simulink model "Koudruped_simcape"  (R2025b)
settings: Solver=VariableStepAuto  StartTime=0.0  StopTime=30  RelTol=1e-2
undefined symbols (not defined in the file or in its folder): fractalcoef, smiData, X, Y, Z
libraries: sm_lib x589, nesl_utility x93, slpidlib x5, mspsensorlib x4, simulink_extras x4, mspfiltlib x3, simulink x2
(part 15 of 16)

== system Koudruped_simcape/quad_step_1_RIGID/govde_step_1_RIGID/A_0002_A_GovdeUst_v11_step_1_RIGID ==
  ReferenceFrame : sm_lib/Frames and Transforms/Reference Frame
  Solid : sm_lib/Body Elements/File Solid  ExtGeomFileName=A-0002-A_GovdeUst v11.step_Varsayılan_sldprt.STEP  UnitType=FromFile  ExtGeomFileUnits=m  StepReaderType=HEX  ExportConvexHullGeometry=off  InertiaType=Custom  BasedOnType=DensityFromFile  Density=1000  DensityUnits=kg/m^3  Mass=smiData.Solid(4).mass  MassUnits=kg  CenterOfMass=smiData.Solid(4).CoM  CenterOfMassUnits=mm  MomentsOfInertia=smiData.Solid(4).MoI  MomentsOfInertiaUnits=kg*mm^2  ProductsOfInertia=smiData.Solid(4).PoI  ProductsOfInertiaUnits=kg*mm^2  GraphicType=FromGeometry  MarkerShape=Sphere  MarkerSize=10  GraphicVisPropType=SimpleVisualProperties  GraphicDiffuseColor=smiData.Solid(4).color  GraphicOpacity=smiData.Solid(4).opacity  GraphicSpecularColor=[0.5 0.5 0.5 1.0]  GraphicAmbientColor=[0.15 0.15 0.15 1.0]  GraphicEmissiveColor=[0.0 0.0 0.0 1.0]  GraphicShininess=75  DoExposeReferenceFrame=on  SerializedFrames=<Frames/>
  F : PMIOPort  Side=Left
  connections:
  ReferenceFrame/RConn1 -- Solid/RConn1 -- F/RConn1

== system Koudruped_simcape/quad_step_1_RIGID/govde_step_1_RIGID/Arms_step_1_RIGID ==
  ReferenceFrame : sm_lib/Frames and Transforms/Reference Frame
  Transform : sm_lib/Frames and Transforms/Rigid Transform  RotationMethod=ArbitraryAxis  FollAlignAxisA=+X  BaseAlignAxisA=+Y  FollAlignAxisB=+Y  BaseAlignAxisB=+Z  RotationStandardAxis=+Z  RotationAngle=smiData.RigidTransform(1).angle  RotationAngleUnits=rad  RotationArbitraryAxis=smiData.RigidTransform(1).axis  RotationSequenceAxes=FollowerAxes  RotationSequence=XYX  RotationSequenceAngles=[0 0 0]  RotationSequenceAnglesUnits=deg  RotationMatrix=[1 0 0;0 1 0;0 0 1]  Quaternion=[1 0 0 0]  TranslationMethod=Cartesian  TranslationCartesianOffset=smiData.RigidTransform(1).translation  TranslationCartesianOffsetUnits=mm  TranslationStandardAxis=+Z  TranslationStandardOffset=0  TranslationStandardOffsetUnits=m  TranslationROffset=0  TranslationROffsetUnits=m  TranslationThetaOffset=0  TranslationThetaOffsetUnits=deg  TranslationZOffset=0  TranslationZOffsetUnits=m
  Transform1 : sm_lib/Frames and Transforms/Rigid Transform  RotationMethod=ArbitraryAxis  FollAlignAxisA=+X  BaseAlignAxisA=+Y  FollAlignAxisB=+Y  BaseAlignAxisB=+Z  RotationStandardAxis=+Z  RotationAngle=smiData.RigidTransform(2).angle  RotationAngleUnits=rad  RotationArbitraryAxis=smiData.RigidTransform(2).axis  RotationSequenceAxes=FollowerAxes  RotationSequence=XYX  RotationSequenceAngles=[0 0 0]  RotationSequenceAnglesUnits=deg  RotationMatrix=[1 0 0;0 1 0;0 0 1]  Quaternion=[1 0 0 0]  TranslationMethod=Cartesian  TranslationCartesianOffset=smiData.RigidTransform(2).translation  TranslationCartesianOffsetUnits=mm  TranslationStandardAxis=+Z  TranslationStandardOffset=0  TranslationStandardOffsetUnits=m  TranslationROffset=0  TranslationROffsetUnits=m  TranslationThetaOffset=0  TranslationThetaOffsetUnits=deg  TranslationZOffset=0  TranslationZOffsetUnits=m
  arm_step_1_RIGID : Subsystem
  F : PMIOPort  Side=Left
  connections:
  Transform/RConn1 -- arm_step_1_RIGID/LConn1
  ReferenceFrame/RConn1 -- Transform/LConn1 -- Transform1/RConn1
  Transform1/LConn1 -- F/RConn1

== system Koudruped_simcape/quad_step_1_RIGID/govde_step_1_RIGID/Eklemler_step_1_RIGID ==
  A_0005_AC_ServoYatagi_sol_v15_step_1_RIGID : Subsystem
  ReferenceFrame : sm_lib/Frames and Transforms/Reference Frame
  Transform : sm_lib/Frames and Transforms/Rigid Transform  RotationMethod=ArbitraryAxis  FollAlignAxisA=+X  BaseAlignAxisA=+Y  FollAlignAxisB=+Y  BaseAlignAxisB=+Z  RotationStandardAxis=+Z  RotationAngle=smiData.RigidTransform(3).angle  RotationAngleUnits=rad  RotationArbitraryAxis=smiData.RigidTransform(3).axis  RotationSequenceAxes=FollowerAxes  RotationSequence=XYX  RotationSequenceAngles=[0 0 0]  RotationSequenceAnglesUnits=deg  RotationMatrix=[1 0 0;0 1 0;0 0 1]  Quaternion=[1 0 0 0]  TranslationMethod=Cartesian  TranslationCartesianOffset=smiData.RigidTransform(3).translation  TranslationCartesianOffsetUnits=mm  TranslationStandardAxis=+Z  TranslationStandardOffset=0  TranslationStandardOffsetUnits=m  TranslationROffset=0  TranslationROffsetUnits=m  TranslationThetaOffset=0  TranslationThetaOffsetUnits=deg  TranslationZOffset=0  TranslationZOffsetUnits=m
  Transform1 : sm_lib/Frames and Transforms/Rigid Transform  RotationMethod=ArbitraryAxis  FollAlignAxisA=+X  BaseAlignAxisA=+Y  FollAlignAxisB=+Y  BaseAlignAxisB=+Z  RotationStandardAxis=+Z  RotationAngle=smiData.RigidTransform(4).angle  RotationAngleUnits=rad  RotationArbitraryAxis=smiData.RigidTransform(4).axis  RotationSequenceAxes=FollowerAxes  RotationSequence=XYX  RotationSequenceAngles=[0 0 0]  RotationSequenceAnglesUnits=deg  RotationMatrix=[1 0 0;0 1 0;0 0 1]  Quaternion=[1 0 0 0]  TranslationMethod=Cartesian  TranslationCartesianOffset=smiData.RigidTransform(4).translation  TranslationCartesianOffsetUnits=mm  TranslationStandardAxis=+Z  TranslationStandardOffset=0  TranslationStandardOffsetUnits=m  TranslationROffset=0  TranslationROffsetUnits=m  TranslationThetaOffset=0  TranslationThetaOffsetUnits=deg  TranslationZOffset=0  TranslationZOffsetUnits=m
  F : PMIOPort  Side=Left
  connections:
  A_0005_AC_ServoYatagi_sol_v15_step_1_RIGID/LConn1 -- Transform/RConn1
  ReferenceFrame/RConn1 -- Transform/LConn1 -- Transform1/RConn1
  Transform1/LConn1 -- F/RConn1

== system Koudruped_simcape/quad_step_1_RIGID/ön takım/ön takım ==
  ReferenceFrame : sm_lib/Frames and Transforms/Reference Frame
  Transform : sm_lib/Frames and Transforms/Rigid Transform  RotationMethod=ArbitraryAxis  FollAlignAxisA=+X  BaseAlignAxisA=+Y  FollAlignAxisB=+Y  BaseAlignAxisB=+Z  RotationStandardAxis=+Z  RotationAngle=smiData.RigidTransform(8).angle  RotationAngleUnits=rad  RotationArbitraryAxis=smiData.RigidTransform(8).axis  RotationSequenceAxes=FollowerAxes  RotationSequence=XYX  RotationSequenceAngles=[0 0 0]  RotationSequenceAnglesUnits=deg  RotationMatrix=[1 0 0;0 1 0;0 0 1]  Quaternion=[1 0 0 0]  TranslationMethod=Cartesian  TranslationCartesianOffset=smiData.RigidTransform(8).translation  TranslationCartesianOffsetUnits=mm  TranslationStandardAxis=+Z  TranslationStandardOffset=0  TranslationStandardOffsetUnits=m  TranslationROffset=0  TranslationROffsetUnits=m  TranslationThetaOffset=0  TranslationThetaOffsetUnits=deg  TranslationZOffset=0  TranslationZOffsetUnits=m
  Transform1 : sm_lib/Frames and Transforms/Rigid Transform  RotationMethod=ArbitraryAxis  FollAlignAxisA=+X  BaseAlignAxisA=+Y  FollAlignAxisB=+Y  BaseAlignAxisB=+Z  RotationStandardAxis=+Z  RotationAngle=smiData.RigidTransform(9).angle  RotationAngleUnits=rad  RotationArbitraryAxis=smiData.RigidTransform(9).axis  RotationSequenceAxes=FollowerAxes  RotationSequence=XYX  RotationSequenceAngles=[0 0 0]  RotationSequenceAnglesUnits=deg  RotationMatrix=[1 0 0;0 1 0;0 0 1]  Quaternion=[1 0 0 0]  TranslationMethod=Cartesian  TranslationCartesianOffset=smiData.RigidTransform(9).translation  TranslationCartesianOffsetUnits=mm  TranslationStandardAxis=+Z  TranslationStandardOffset=0  TranslationStandardOffsetUnits=m  TranslationROffset=0  TranslationROffsetUnits=m  TranslationThetaOffset=0  TranslationThetaOffsetUnits=deg  TranslationZOffset=0  TranslationZOffsetUnits=m
  Transform2 : sm_lib/Frames and Transforms/Rigid Transform  RotationMethod=ArbitraryAxis  FollAlignAxisA=+X  BaseAlignAxisA=+Y  FollAlignAxisB=+Y  BaseAlignAxisB=+Z  RotationStandardAxis=+Z  RotationAngle=smiData.RigidTransform(10).angle  RotationAngleUnits=rad  RotationArbitraryAxis=smiData.RigidTransform(10).axis  RotationSequenceAxes=FollowerAxes  RotationSequence=XYX  RotationSequenceAngles=[0 0 0]  RotationSequenceAnglesUnits=deg  RotationMatrix=[1 0 0;0 1 0;0 0 1]  Quaternion=[1 0 0 0]  TranslationMethod=Cartesian  TranslationCartesianOffset=smiData.RigidTransform(10).translation  TranslationCartesianOffsetUnits=mm  TranslationStandardAxis=+Z  TranslationStandardOffset=0  TranslationStandardOffsetUnits=m  TranslationROffset=0  TranslationROffsetUnits=m  TranslationThetaOffset=0  TranslationThetaOffsetUnits=deg  TranslationZOffset=0  TranslationZOffsetUnits=m
  Transform3 : sm_lib/Frames and Transforms/Rigid Transform  RotationMethod=ArbitraryAxis  FollAlignAxisA=+X  BaseAlignAxisA=+Y  FollAlignAxisB=+Y  BaseAlignAxisB=+Z  RotationStandardAxis=+Z  RotationAngle=smiData.RigidTransform(11).angle  RotationAngleUnits=rad  RotationArbitraryAxis=smiData.RigidTransform(11).axis  RotationSequenceAxes=FollowerAxes  RotationSequence=XYX  RotationSequenceAngles=[0 0 0]  RotationSequenceAnglesUnits=deg  RotationMatrix=[1 0 0;0 1 0;0 0 1]  Quaternion=[1 0 0 0]  TranslationMethod=Cartesian  TranslationCartesianOffset=smiData.RigidTransform(11).translation  TranslationCartesianOffsetUnits=mm  TranslationStandardAxis=+Z  TranslationStandardOffset=0  TranslationStandardOffsetUnits=m  TranslationROffset=0  TranslationROffsetUnits=m  TranslationThetaOffset=0  TranslationThetaOffsetUnits=deg  TranslationZOffset=0  TranslationZOffsetUnits=m
  arm_v2_1_step_1_RIGID : Subsystem
  ön alt : Subsystem
  ön üst : Subsystem
  F : PMIOPort  Side=Left
  connections:
  ön alt/LConn1 -- Transform/RConn1
  Transform1/RConn1 -- arm_v2_1_step_1_RIGID/LConn1
  Transform2/RConn1 -- ön üst/LConn1
  ReferenceFrame/RConn1 -- Transform1/LConn1 -- Transform2/LConn1 -- Transform/LConn1 -- Transform3/RConn1
  Transform3/LConn1 -- F/RConn1

== system Koudruped_simcape/quad_step_1_RIGID/govde_step_1_RIGID/Arms_step_1_RIGID/arm_step_1_RIGID ==
  ReferenceFrame : sm_lib/Frames and Transforms/Reference Frame
  Solid : sm_lib/Body Elements/File Solid  ExtGeomFileName=arm.step_Varsayılan_sldprt.STEP  UnitType=FromFile  ExtGeomFileUnits=m  StepReaderType=HEX  ExportConvexHullGeometry=off  InertiaType=Custom  BasedOnType=DensityFromFile  Density=1000  DensityUnits=kg/m^3  Mass=smiData.Solid(1).mass  MassUnits=kg  CenterOfMass=smiData.Solid(1).CoM  CenterOfMassUnits=mm  MomentsOfInertia=smiData.Solid(1).MoI  MomentsOfInertiaUnits=kg*mm^2  ProductsOfInertia=smiData.Solid(1).PoI  ProductsOfInertiaUnits=kg*mm^2  GraphicType=FromGeometry  MarkerShape=Sphere  MarkerSize=10  GraphicVisPropType=SimpleVisualProperties  GraphicDiffuseColor=smiData.Solid(1).color  GraphicOpacity=smiData.Solid(1).opacity  GraphicSpecularColor=[0.5 0.5 0.5 1.0]  GraphicAmbientColor=[0.15 0.15 0.15 1.0]  GraphicEmissiveColor=[0.0 0.0 0.0 1.0]  GraphicShininess=75  DoExposeReferenceFrame=on  SerializedFrames=<Frames/>
  F : PMIOPort  Side=Left
  connections:
  ReferenceFrame/RConn1 -- Solid/RConn1 -- F/RConn1

== system Koudruped_simcape/quad_step_1_RIGID/govde_step_1_RIGID/Eklemler_step_1_RIGID/A_0005_AC_ServoYatagi_sol_v15_step_1_RIGID ==
  ReferenceFrame : sm_lib/Frames and Transforms/Reference Frame
  Solid : sm_lib/Body Elements/File Solid  ExtGeomFileName=A_0005_AC_ServoYatagi_sol v15.step_Varsayılan_sldprt.STEP  UnitType=FromFile  ExtGeomFileUnits=m  StepReaderType=HEX  ExportConvexHullGeometry=off  InertiaType=Custom  BasedOnType=DensityFromFile  Density=1000  DensityUnits=kg/m^3  Mass=smiData.Solid(2).mass  MassUnits=kg  CenterOfMass=smiData.Solid(2).CoM  CenterOfMassUnits=mm  MomentsOfInertia=smiData.Solid(2).MoI  MomentsOfInertiaUnits=kg*mm^2  ProductsOfInertia=smiData.Solid(2).PoI  ProductsOfInertiaUnits=kg*mm^2  GraphicType=FromGeometry  MarkerShape=Sphere  MarkerSize=10  GraphicVisPropType=SimpleVisualProperties  GraphicDiffuseColor=smiData.Solid(2).color  GraphicOpacity=smiData.Solid(2).opacity  GraphicSpecularColor=[0.5 0.5 0.5 1.0]  GraphicAmbientColor=[0.15 0.15 0.15 1.0]  GraphicEmissiveColor=[0.0 0.0 0.0 1.0]  GraphicShininess=75  DoExposeReferenceFrame=on  SerializedFrames=<Frames/>
  F : PMIOPort  Side=Left
  connections:
  ReferenceFrame/RConn1 -- Solid/RConn1 -- F/RConn1

== system Koudruped_simcape/quad_step_1_RIGID/ön takım/ön takım/arm_v2_1_step_1_RIGID ==
  ReferenceFrame : sm_lib/Frames and Transforms/Reference Frame
  Solid : sm_lib/Body Elements/File Solid  ExtGeomFileName=arm v2 (1).step_Varsayılan_sldprt.STEP  UnitType=FromFile  ExtGeomFileUnits=m  StepReaderType=HEX  ExportConvexHullGeometry=off  InertiaType=Custom  BasedOnType=DensityFromFile  Density=1000  DensityUnits=kg/m^3  Mass=smiData.Solid(6).mass  MassUnits=kg  CenterOfMass=smiData.Solid(6).CoM  CenterOfMassUnits=mm  MomentsOfInertia=smiData.Solid(6).MoI  MomentsOfInertiaUnits=kg*mm^2  ProductsOfInertia=smiData.Solid(6).PoI  ProductsOfInertiaUnits=kg*mm^2  GraphicType=FromGeometry  MarkerShape=Sphere  MarkerSize=10  GraphicVisPropType=SimpleVisualProperties  GraphicDiffuseColor=smiData.Solid(6).color  GraphicOpacity=smiData.Solid(6).opacity  GraphicSpecularColor=[0.5 0.5 0.5 1.0]  GraphicAmbientColor=[0.15 0.15 0.15 1.0]  GraphicEmissiveColor=[0.0 0.0 0.0 1.0]  GraphicShininess=75  DoExposeReferenceFrame=on  SerializedFrames=<Frames/>
  F : PMIOPort  Side=Left
  connections:
  ReferenceFrame/RConn1 -- Solid/RConn1 -- F/RConn1

== system Koudruped_simcape/quad_step_1_RIGID/ön takım/ön takım/ön alt ==
  ReferenceFrame : sm_lib/Frames and Transforms/Reference Frame
  ön alt : sm_lib/Body Elements/File Solid  ExtGeomFileName=Alt Bacak v3.step_Varsayılan_sldprt.STEP  UnitType=FromFile  ExtGeomFileUnits=m  StepReaderType=HEX  ExportConvexHullGeometry=off  InertiaType=Custom  BasedOnType=DensityFromFile  Density=1000  DensityUnits=kg/m^3  Mass=smiData.Solid(5).mass  MassUnits=kg  CenterOfMass=smiData.Solid(5).CoM  CenterOfMassUnits=mm  MomentsOfInertia=smiData.Solid(5).MoI  MomentsOfInertiaUnits=kg*mm^2  ProductsOfInertia=smiData.Solid(5).PoI  ProductsOfInertiaUnits=kg*mm^2  GraphicType=FromGeometry  MarkerShape=Sphere  MarkerSize=10  GraphicVisPropType=SimpleVisualProperties  GraphicDiffuseColor=smiData.Solid(5).color  GraphicOpacity=smiData.Solid(5).opacity  GraphicSpecularColor=[0.5 0.5 0.5 1.0]  GraphicAmbientColor=[0.15 0.15 0.15 1.0]  GraphicEmissiveColor=[0.0 0.0 0.0 1.0]  GraphicShininess=75  DoExposeReferenceFrame=on  SerializedFrames=<Frames/>
  F : PMIOPort  Side=Left
  connections:
  ReferenceFrame/RConn1 -- ön alt/RConn1 -- F/RConn1

== system Koudruped_simcape/quad_step_1_RIGID/ön takım/ön takım/ön üst ==
  ReferenceFrame : sm_lib/Frames and Transforms/Reference Frame
  ön üst : sm_lib/Body Elements/File Solid  ExtGeomFileName=_X_DCst Bacak v3.step_Varsayılan_sldprt.STEP  UnitType=FromFile  ExtGeomFileUnits=m  StepReaderType=HEX  ExportConvexHullGeometry=off  InertiaType=Custom  BasedOnType=DensityFromFile  Density=1000  DensityUnits=kg/m^3  Mass=smiData.Solid(7).mass  MassUnits=kg  CenterOfMass=smiData.Solid(7).CoM  CenterOfMassUnits=mm  MomentsOfInertia=smiData.Solid(7).MoI  MomentsOfInertiaUnits=kg*mm^2  ProductsOfInertia=smiData.Solid(7).PoI  ProductsOfInertiaUnits=kg*mm^2  GraphicType=FromGeometry  MarkerShape=Sphere  MarkerSize=10  GraphicVisPropType=SimpleVisualProperties  GraphicDiffuseColor=smiData.Solid(7).color  GraphicOpacity=smiData.Solid(7).opacity  GraphicSpecularColor=[0.5 0.5 0.5 1.0]  GraphicAmbientColor=[0.15 0.15 0.15 1.0]  GraphicEmissiveColor=[0.0 0.0 0.0 1.0]  GraphicShininess=75  DoExposeReferenceFrame=on  SerializedFrames=<Frames/>
  F : PMIOPort  Side=Left
  connections:
  ReferenceFrame/RConn1 -- ön üst/RConn1 -- F/RConn1

== matlab function Koudruped_simcape/Right Front Step/MATLAB Function12 ==
  data: t input; pos output; phase_offset input; H_hedef input
function pos = fcn(t, phase_offset, H_hedef)
    pos = zeros(3,1); 
    
    % --- PARAMETRELER ---
    T_kalkis = 2.0;      
    T_bekleme = 1.0;     
    T_periyot = 1.0;     
    Duty_Factor = 0.5;   
    
    L_adim = 80;         
    H_adim = 30;         
    H_baslangic = -50;   
    Y_offset = 60;       
    
    % --- DURUM MAKİNESİ ---
    if t < T_kalkis
        z = H_baslangic + (H_hedef - H_baslangic) * (t / T_kalkis);
        x = 0;
        pos = [x; Y_offset; z];
        
    elseif t < (T_kalkis + T_bekleme)
        z = H_hedef;
        x = 0;
        pos = [x; Y_offset; z];
        
    else
        t_yurume = t - (T_kalkis + T_bekleme);
        
        % === FADE-IN (YUMUŞAK BAŞLANGIÇ) ÇARPANI ===
        % İlk 2 saniye boyunca adım boyu ve yüksekliği 0'dan 100%'e çıkar
        T_fade = 2.0; 
        k_amp = min(t_yurume / T_fade, 1.0); 
        
        % O anki aktif adım limitleri
        L_aktif = L_adim * k_amp;
        H_aktif = H_adim * k_amp;
        
        t_norm = mod((t_yurume / T_periyot) + phase_offset, 1.0);
        
        if t_norm < Duty_Factor
            % Swing Phase
            t_swing = t_norm / Duty_Factor; 
            x = -(L_aktif/2) + L_aktif * (t_swing - sin(2*pi*t_swing)/(2*pi));
            z = H_hedef + H_aktif * sin(pi * t_swing); 
        else
            % Stance Phase
            t_stance = (t_norm - Duty_Factor) / (1 - Duty_Factor);
            x_start = L_aktif/2;
            x_end = -(L_aktif/2);
            x = x_start + (x_end - x_start) * ((1 - cos(pi * t_stance)) / 2);
            z = H_hedef;
        end
        
        pos = [x; Y_offset; z];
    end
end

== matlab function Koudruped_simcape/Right Front Step/MATLAB Function13 ==
  data: pos input; angles output
function angles = inverse(pos)
    x = pos(1); y = pos(2); z = pos(3);
    
    % --- PARAMETRELER (Senin değerlerin) ---
    L1 = 44.41; a1 = 24.51; L2 = 100; L3 = 100;
    
    % --- 1. OMUZ (ROLL) ---
    % Omuzun dışa doğru açılması için atan2 parametrelerini kontrol et
    % Eğer omuz içeri katlanıyorsa 'y' yerine '-y' deneyebilirsin
    theta1_rad = atan2(y, -z) - atan2(L1, sqrt(y^2 + z^2 - L1^2));

    % --- 2. YARDIMCI KOORDİNATLAR ---
    % Bacak düzlemindeki izdüşüm
    r = sqrt(y^2 + z^2 - L1^2) - a1;
    % Yeni düzlemde hedef noktası (x, r)
    dist_sq = x^2 + r^2;
    dist = sqrt(dist_sq);

    % --- 3. DİZ (KNEE) ---
    cos_phi = (L2^2 + L3^2 - dist_sq) / (2 * L2 * L3);
    cos_phi = min(max(cos_phi, -1), 1); % Sayısal koruma
    phi = acos(cos_phi);
    % theta3'ü pozitif yaparsan diz ters yöne kırılır
    theta3_rad = -(pi - phi); 

    % --- 4. KALÇA (PITCH) ---
    alpha = atan2(x, r);
    beta = acos((L2^2 + dist_sq - L3^2) / (2 * L2 * dist));
    theta2_rad = alpha + beta;

    % RAD -> DEG
    angles = [theta1_rad; theta2_rad; theta3_rad] * (180/pi);
end

== matlab function Koudruped_simcape/Sol Ön Adım1/MATLAB Function1 ==
  data: t input; pos output; phase_offset input
function pos = fcn(t, phase_offset)
    pos = zeros(3,1); 
    
    % --- PARAMETRELER ---
    T_kalkis = 2.0;      
    T_bekleme = 1.0;     
    T_periyot = 2.0;     % Walk gait daha yavaştır, stabilite için 1.0'dan 2.0'a çıkarıldı.
    Swing_Ratio = 0.25;  % Walk gait için havada kalma süresi periyodun %25'i olmalı.
    
    L_adim = 80;         
    H_adim = 30;         
    H_baslangic = -50;   
    H_hedef = -130;
    Y_offset = 60;       
    
    % --- DURUM MAKİNESİ ---
    if t < T_kalkis
        z = H_baslangic + (H_hedef - H_baslangic) * (t / T_kalkis);
        x = 0;
        pos = [x; Y_offset; z];
        
    elseif t < (T_kalkis + T_bekleme)
        z = H_hedef-2;
        x = 0;
        pos = [x; Y_offset; z];
        
    else
        t_yurume = t - (T_kalkis + T_bekleme);
        
        % === FADE-IN (YUMUŞAK BAŞLANGIÇ) ÇARPANI ===
        T_fade = 2.0; 
        k_amp = min(t_yurume / T_fade, 1.0); 
        
        L_aktif = L_adim * k_amp;
        H_aktif = H_adim * k_amp;
        
        t_norm = mod((t_yurume / T_periyot) + phase_offset, 1.0);
        
        if t_norm < Swing_Ratio
            % Swing Phase (Havada)
            t_swing = t_norm / Swing_Ratio; 
            x = -(L_aktif/2) + L_aktif * (t_swing - sin(2*pi*t_swing)/(2*pi));
            z = H_hedef + H_aktif * sin(pi * t_swing); 
        else
            % Stance Phase (Yerde İtme)
            t_stance = (t_norm - Swing_Ratio) / (1 - Swing_Ratio);
            x_start = L_aktif/2;
            x_end = -(L_aktif/2);
            x = x_start + (x_end - x_start) * ((1 - cos(pi * t_stance)) / 2);
            z = H_hedef;
        end
        
        pos = [x; Y_offset; z];
    end
end

== matlab function Koudruped_simcape/Sol Ön Adım1/MATLAB Function2 ==
  data: pos input; angles output
function angles = inverse(pos)
    x = pos(1); y = pos(2); z = pos(3);
    
    % --- PARAMETRELER (Senin değerlerin) ---
    L1 = 44.41; a1 = 24.51; L2 = 100; L3 = 102.5;
    
    % --- 1. OMUZ (ROLL) ---
    % Omuzun dışa doğru açılması için atan2 parametrelerini kontrol et
    % Eğer omuz içeri katlanıyorsa 'y' yerine '-y' deneyebilirsin
    theta1_rad = atan2(y, -z) - atan2(L1, sqrt(y^2 + z^2 - L1^2));

    % --- 2. YARDIMCI KOORDİNATLAR ---
    % Bacak düzlemindeki izdüşüm
    r = sqrt(y^2 + z^2 - L1^2) - a1;
    % Yeni düzlemde hedef noktası (x, r)
    dist_sq = x^2 + r^2;
    dist = sqrt(dist_sq);

    % --- 3. DİZ (KNEE) ---
    cos_phi = (L2^2 + L3^2 - dist_sq) / (2 * L2 * L3);
    cos_phi = min(max(cos_phi, -1), 1); % Sayısal koruma
    phi = acos(cos_phi);
    % theta3'ü pozitif yaparsan diz ters yöne kırılır
    theta3_rad = -(pi - phi); 

    % --- 4. KALÇA (PITCH) ---
    alpha = atan2(x, r);
    beta = acos((L2^2 + dist_sq - L3^2) / (2 * L2 * dist));
    theta2_rad = alpha + beta;

    % RAD -> DEG
    angles = [theta1_rad; theta2_rad; theta3_rad] * (180/pi);
end

== matlab function Koudruped_simcape/Sağ Arka Adım2/MATLAB Function1 ==
  data: t input; pos output; phase_offset input; H_hedef input
function pos = fcn(t, phase_offset, H_hedef)
    pos = zeros(3,1); 
    
    % --- PARAMETRELER ---
    T_kalkis = 2.0;      
    T_bekleme = 1.0;     
    T_periyot = 1.0;     
    Duty_Factor = 0.5;   
    
    L_adim = 80;         
    H_adim = 30;         
    H_baslangic = -50;   
    Y_offset = 60;       
    
    % --- DURUM MAKİNESİ ---
    if t < T_kalkis
        z = H_baslangic + (H_hedef - H_baslangic) * (t / T_kalkis);
        x = 0;
        pos = [x; Y_offset; z];
        
    elseif t < (T_kalkis + T_bekleme)
        z = H_hedef;
        x = 0;
        pos = [x; Y_offset; z];
        
    else
        t_yurume = t - (T_kalkis + T_bekleme);
        
        % === FADE-IN (YUMUŞAK BAŞLANGIÇ) ÇARPANI ===
        % İlk 2 saniye boyunca adım boyu ve yüksekliği 0'dan 100%'e çıkar
        T_fade = 2.0; 
        k_amp = min(t_yurume / T_fade, 1.0); 
        
        % O anki aktif adım limitleri
        L_aktif = L_adim * k_amp;
        H_aktif = H_adim * k_amp;
        
        t_norm = mod((t_yurume / T_periyot) + phase_offset, 1.0);
        
        if t_norm < Duty_Factor
            % Swing Phase
            t_swing = t_norm / Duty_Factor; 
            x = -(L_aktif/2) + L_aktif * (t_swing - sin(2*pi*t_swing)/(2*pi));
            z = H_hedef + H_aktif * sin(pi * t_swing); 
        else
            % Stance Phase
            t_stance = (t_norm - Duty_Factor) / (1 - Duty_Factor);
            x_start = L_aktif/2;
            x_end = -(L_aktif/2);
            x = x_start + (x_end - x_start) * ((1 - cos(pi * t_stance)) / 2);
            z = H_hedef;
        end
        
        pos = [x; Y_offset; z];
    end
end

== matlab function Koudruped_simcape/Sağ Arka Adım2/MATLAB Function2 ==
  data: pos input; angles output
function angles = inverse(pos)
    x = pos(1); y = pos(2); z = pos(3);
    
    % --- PARAMETRELER (Senin değerlerin) ---
    L1 = 44.41; a1 = 24.51; L2 = 100; L3 = 100;
    
    % --- 1. OMUZ (ROLL) ---
    % Omuzun dışa doğru açılması için atan2 parametrelerini kontrol et
    % Eğer omuz içeri katlanıyorsa 'y' yerine '-y' deneyebilirsin
    theta1_rad = atan2(y, -z) - atan2(L1, sqrt(y^2 + z^2 - L1^2));

    % --- 2. YARDIMCI KOORDİNATLAR ---
    % Bacak düzlemindeki izdüşüm
    r = sqrt(y^2 + z^2 - L1^2) - a1;
    % Yeni düzlemde hedef noktası (x, r)
    dist_sq = x^2 + r^2;
    dist = sqrt(dist_sq);

    % --- 3. DİZ (KNEE) ---
    cos_phi = (L2^2 + L3^2 - dist_sq) / (2 * L2 * L3);
    cos_phi = min(max(cos_phi, -1), 1); % Sayısal koruma
    phi = acos(cos_phi);
    % theta3'ü pozitif yaparsan diz ters yöne kırılır
    theta3_rad = -(pi - phi); 

    % --- 4. KALÇA (PITCH) ---
    alpha = atan2(x, r);
    beta = acos((L2^2 + dist_sq - L3^2) / (2 * L2 * dist));
    theta2_rad = alpha + beta;

    % RAD -> DEG
    angles = [theta1_rad; theta2_rad; theta3_rad] * (180/pi);
end

== matlab function Koudruped_simcape/Sağ Ön Adım2/MATLAB Function12 ==
  data: t input; pos output; phase_offset input; H_hedef input
function pos = fcn(t, phase_offset, H_hedef)
    pos = zeros(3,1); 
    
    % --- PARAMETRELER ---
    T_kalkis = 2.0;      
    T_bekleme = 1.0;     
    T_periyot = 1.0;     
    Duty_Factor = 0.5;   
    
    L_adim = 80;         
    H_adim = 30;         
    H_baslangic = -50;   
    Y_offset = 60;       
    
    % --- DURUM MAKİNESİ ---
    if t < T_kalkis
        z = H_baslangic + (H_hedef - H_baslangic) * (t / T_kalkis);
        x = 0;
        pos = [x; Y_offset; z];
        
    elseif t < (T_kalkis + T_bekleme)
        z = H_hedef;
        x = 0;
        pos = [x; Y_offset; z];
        
    else
        t_yurume = t - (T_kalkis + T_bekleme);
        
        % === FADE-IN (YUMUŞAK BAŞLANGIÇ) ÇARPANI ===
        % İlk 2 saniye boyunca adım boyu ve yüksekliği 0'dan 100%'e çıkar
        T_fade = 2.0; 
        k_amp = min(t_yurume / T_fade, 1.0); 
        
        % O anki aktif adım limitleri
        L_aktif = L_adim * k_amp;
        H_aktif = H_adim * k_amp;
        
        t_norm = mod((t_yurume / T_periyot) + phase_offset, 1.0);
        
        if t_norm < Duty_Factor
            % Swing Phase
            t_swing = t_norm / Duty_Factor; 
            x = -(L_aktif/2) + L_aktif * (t_swing - sin(2*pi*t_swing)/(2*pi));
            z = H_hedef + H_aktif * sin(pi * t_swing); 
        else
            % Stance Phase
            t_stance = (t_norm - Duty_Factor) / (1 - Duty_Factor);
            x_start = L_aktif/2;
            x_end = -(L_aktif/2);
            x = x_start + (x_end - x_start) * ((1 - cos(pi * t_stance)) / 2);
            z = H_hedef;
        end
        
        pos = [x; Y_offset; z];
    end
end

== matlab function Koudruped_simcape/Sağ Ön Adım2/MATLAB Function13 ==
  data: pos input; angles output
function angles = inverse(pos)
    x = pos(1); y = pos(2); z = pos(3);
    
    % --- PARAMETRELER (Senin değerlerin) ---
    L1 = 44.41; a1 = 24.51; L2 = 100; L3 = 100;
    
    % --- 1. OMUZ (ROLL) ---
    % Omuzun dışa doğru açılması için atan2 parametrelerini kontrol et
    % Eğer omuz içeri katlanıyorsa 'y' yerine '-y' deneyebilirsin
    theta1_rad = atan2(y, -z) - atan2(L1, sqrt(y^2 + z^2 - L1^2));

    % --- 2. YARDIMCI KOORDİNATLAR ---
    % Bacak düzlemindeki izdüşüm
    r = sqrt(y^2 + z^2 - L1^2) - a1;
    % Yeni düzlemde hedef noktası (x, r)
    dist_sq = x^2 + r^2;
    dist = sqrt(dist_sq);

    % --- 3. DİZ (KNEE) ---
    cos_phi = (L2^2 + L3^2 - dist_sq) / (2 * L2 * L3);
    cos_phi = min(max(cos_phi, -1), 1); % Sayısal koruma
    phi = acos(cos_phi);
    % theta3'ü pozitif yaparsan diz ters yöne kırılır
    theta3_rad = -(pi - phi); 

    % --- 4. KALÇA (PITCH) ---
    alpha = atan2(x, r);
    beta = acos((L2^2 + dist_sq - L3^2) / (2 * L2 * dist));
    theta2_rad = alpha + beta;

    % RAD -> DEG
    angles = [theta1_rad; theta2_rad; theta3_rad] * (180/pi);
end

== matlab function Koudruped_simcape/Sol Arka Adım2/MATLAB Function1 ==
  data: t input; pos output; phase_offset input; H_hedef input
function pos = fcn(t, phase_offset, H_hedef)
    pos = zeros(3,1); 
    
    % --- PARAMETRELER ---
    T_kalkis = 2.0;      
    T_bekleme = 1.0;     
    T_periyot = 1.0;     
    Duty_Factor = 0.5;   
    
    L_adim = 80;         
    H_adim = 30;         
    H_baslangic = -50;   
    Y_offset = 60;       
    
    % --- DURUM MAKİNESİ ---
    if t < T_kalkis
        z = H_baslangic + (H_hedef - H_baslangic) * (t / T_kalkis);
        x = 0;
        pos = [x; Y_offset; z];
        
    elseif t < (T_kalkis + T_bekleme)
        z = H_hedef;
        x = 0;
        pos = [x; Y_offset; z];
        
    else
        t_yurume = t - (T_kalkis + T_bekleme);
        
        % === FADE-IN (YUMUŞAK BAŞLANGIÇ) ÇARPANI ===
        % İlk 2 saniye boyunca adım boyu ve yüksekliği 0'dan 100%'e çıkar
        T_fade = 2.0; 
        k_amp = min(t_yurume / T_fade, 1.0); 
        
        % O anki aktif adım limitleri
        L_aktif = L_adim * k_amp;
        H_aktif = H_adim * k_amp;
        
        t_norm = mod((t_yurume / T_periyot) + phase_offset, 1.0);
        
        if t_norm < Duty_Factor
            % Swing Phase
            t_swing = t_norm / Duty_Factor; 
            x = -(L_aktif/2) + L_aktif * (t_swing - sin(2*pi*t_swing)/(2*pi));
            z = H_hedef + H_aktif * sin(pi * t_swing); 
        else
            % Stance Phase
            t_stance = (t_norm - Duty_Factor) / (1 - Duty_Factor);
            x_start = L_aktif/2;
            x_end = -(L_aktif/2);
            x = x_start + (x_end - x_start) * ((1 - cos(pi * t_stance)) / 2);
            z = H_hedef;
        end
        
        pos = [x; Y_offset; z];
    end
end

== matlab function Koudruped_simcape/Sol Arka Adım2/MATLAB Function2 ==
  data: pos input; angles output
function angles = inverse(pos)
    x = pos(1); y = pos(2); z = pos(3);
    
    % --- PARAMETRELER (Senin değerlerin) ---
    L1 = 44.41; a1 = 24.51; L2 = 100; L3 = 100;
    
    % --- 1. OMUZ (ROLL) ---
    % Omuzun dışa doğru açılması için atan2 parametrelerini kontrol et
    % Eğer omuz içeri katlanıyorsa 'y' yerine '-y' deneyebilirsin
    theta1_rad = atan2(y, -z) - atan2(L1, sqrt(y^2 + z^2 - L1^2));

    % --- 2. YARDIMCI KOORDİNATLAR ---
    % Bacak düzlemindeki izdüşüm
    r = sqrt(y^2 + z^2 - L1^2) - a1;
    % Yeni düzlemde hedef noktası (x, r)
    dist_sq = x^2 + r^2;
    dist = sqrt(dist_sq);

    % --- 3. DİZ (KNEE) ---
    cos_phi = (L2^2 + L3^2 - dist_sq) / (2 * L2 * L3);
    cos_phi = min(max(cos_phi, -1), 1); % Sayısal koruma
    phi = acos(cos_phi);
    % theta3'ü pozitif yaparsan diz ters yöne kırılır
    theta3_rad = -(pi - phi); 

    % --- 4. KALÇA (PITCH) ---
    alpha = atan2(x, r);
    beta = acos((L2^2 + dist_sq - L3^2) / (2 * L2 * dist));
    theta2_rad = alpha + beta;

    % RAD -> DEG
    angles = [theta1_rad; theta2_rad; theta3_rad] * (180/pi);
end

== matlab function Koudruped_simcape/Right Back Step/MATLAB Function2 ==
  data: pos input; angles output
function angles = inverse(pos)
    x = pos(1); y = pos(2); z = pos(3);
    
    % --- PARAMETRELER (Senin değerlerin) ---
    L1 = 44.41; a1 = 24.51; L2 = 100; L3 = 100;
    
    % --- 1. OMUZ (ROLL) ---
    % Omuzun dışa doğru açılması için atan2 parametrelerini kontrol et
    % Eğer omuz içeri katlanıyorsa 'y' yerine '-y' deneyebilirsin
    theta1_rad = atan2(y, -z) - atan2(L1, sqrt(y^2 + z^2 - L1^2));

    % --- 2. YARDIMCI KOORDİNATLAR ---
    % Bacak düzlemindeki izdüşüm
    r = sqrt(y^2 + z^2 - L1^2) - a1;
    % Yeni düzlemde hedef noktası (x, r)
    dist_sq = x^2 + r^2;
    dist = sqrt(dist_sq);

    % --- 3. DİZ (KNEE) ---
    cos_phi = (L2^2 + L3^2 - dist_sq) / (2 * L2 * L3);
    cos_phi = min(max(cos_phi, -1), 1); % Sayısal koruma
    phi = acos(cos_phi);
    % theta3'ü pozitif yaparsan diz ters yöne kırılır
    theta3_rad = -(pi - phi); 

    % --- 4. KALÇA (PITCH) ---
    alpha = atan2(x, r);
    beta = acos((L2^2 + dist_sq - L3^2) / (2 * L2 * dist));
    theta2_rad = alpha + beta;

    % RAD -> DEG
    angles = [theta1_rad; theta2_rad; theta3_rad] * (180/pi);
end

== matlab function Koudruped_simcape/Sol Ön Adım2/MATLAB Function1 ==
  data: t input; pos output; phase_offset input; H_hedef input
function pos = fcn(t, phase_offset, H_hedef)
    pos = zeros(3,1); 
    
    % --- PARAMETRELER ---
    T_kalkis = 2.0;      
    T_bekleme = 1.0;     
    T_periyot = 1.0;     
    Duty_Factor = 0.5;   
    
    L_adim = 80;         
    H_adim = 30;         
    H_baslangic = -50;   
    Y_offset = 60;       
    
    % --- DURUM MAKİNESİ ---
    if t < T_kalkis
        z = H_baslangic + (H_hedef - H_baslangic) * (t / T_kalkis);
        x = 0;
        pos = [x; Y_offset; z];
        
    elseif t < (T_kalkis + T_bekleme)
        z = H_hedef;
        x = 0;
        pos = [x; Y_offset; z];
        
    else
        t_yurume = t - (T_kalkis + T_bekleme);
        
        % === FADE-IN (YUMUŞAK BAŞLANGIÇ) ÇARPANI ===
        % İlk 2 saniye boyunca adım boyu ve yüksekliği 0'dan 100%'e çıkar
        T_fade = 2.0; 
        k_amp = min(t_yurume / T_fade, 1.0); 
        
        % O anki aktif adım limitleri
        L_aktif = L_adim * k_amp;
        H_aktif = H_adim * k_amp;
        
        t_norm = mod((t_yurume / T_periyot) + phase_offset, 1.0);
        
        if t_norm < Duty_Factor
            % Swing Phase
            t_swing = t_norm / Duty_Factor; 
            x = -(L_aktif/2) + L_aktif * (t_swing - sin(2*pi*t_swing)/(2*pi));
            z = H_hedef + H_aktif * sin(pi * t_swing); 
        else
            % Stance Phase
            t_stance = (t_norm - Duty_Factor) / (1 - Duty_Factor);
            x_start = L_aktif/2;
            x_end = -(L_aktif/2);
            x = x_start + (x_end - x_start) * ((1 - cos(pi * t_stance)) / 2);
            z = H_hedef;
        end
        
        pos = [x; Y_offset; z];
    end
end

== matlab function Koudruped_simcape/Sol Ön Adım2/MATLAB Function2 ==
  data: pos input; angles output
function angles = inverse(pos)
    x = pos(1); y = pos(2); z = pos(3);
    
    % --- PARAMETRELER (Senin değerlerin) ---
    L1 = 44.41; a1 = 24.51; L2 = 100; L3 = 100;
    
    % --- 1. OMUZ (ROLL) ---
    theta1_rad = atan2(y, -z) - atan2(L1, sqrt(y^2 + z^2 - L1^2));

    % --- 2. YARDIMCI KOORDİNATLAR ---
    % Bacak düzlemindeki izdüşüm
    r = sqrt(y^2 + z^2 - L1^2) - a1;
    % Yeni düzlemde hedef noktası (x, r)
    dist_sq = x^2 + r^2;
    dist = sqrt(dist_sq);

    % --- 3. DİZ (KNEE) ---
    cos_phi = (L2^2 + L3^2 - dist_sq) / (2 * L2 * L3);
    cos_phi = min(max(cos_phi, -1), 1); % Sayısal koruma
    phi = acos(cos_phi);
    % theta3'ü pozitif yaparsan diz ters yöne kırılır
    theta3_rad = -(pi - phi); 

    % --- 4. KALÇA (PITCH) ---
    alpha = atan2(x, r);
    beta = acos((L2^2 + dist_sq - L3^2) / (2 * L2 * dist));
    theta2_rad = alpha + beta;

    % RAD -> DEG
    angles = [theta1_rad; theta2_rad; theta3_rad] * (180/pi);
end

== matlab function Koudruped_simcape/Left Back Step1/MATLAB Function1 ==
  data: t input; pos output; phase_offset input; H_hedef input
function pos = fcn(t, phase_offset, H_hedef)
    pos = zeros(3,1); 
    
    % === 1. ADIM: BU BACAK İÇİN DEĞERLERİ YUKARIDAKİ LİSTEYE GÖRE GİR ===
    X_merkez = -40;       % Ön için 0, Arka için -40
    Y_offset = 44.41;   % Sol için 44.41, Sağ için -44.41
    
    % --- PARAMETRELER ---
    T_kalkis = 2.0;      
    H_baslangic = -190;  
    
    % --- DURUM MAKİNESİ (Sadece Z ekseni hareket eder) ---
    if t < T_kalkis
        z = H_baslangic + (H_hedef - H_baslangic) * (t / T_kalkis);
    else
        z = H_hedef;
    end
    
    x = X_merkez;
    y = Y_offset;
    
    pos = [x; y; z];
end

== matlab function Koudruped_simcape/Left Back Step1/MATLAB Function2 ==
  data: pos input; angles output
function angles = inverse(pos)
    x = pos(1); y = pos(2); z = pos(3);
    
    % --- PARAMETRELER (Senin değerlerin) ---
    L1 = 44.41; a1 = 24.51; L2 = 100; L3 = 100;
    
    % --- 1. OMUZ (ROLL) ---
    % Omuzun dışa doğru açılması için atan2 parametrelerini kontrol et
    % Eğer omuz içeri katlanıyorsa 'y' yerine '-y' deneyebilirsin
    theta1_rad = atan2(y, -z) - atan2(L1, sqrt(y^2 + z^2 - L1^2));

    % --- 2. YARDIMCI KOORDİNATLAR ---
    % Bacak düzlemindeki izdüşüm
    r = sqrt(y^2 + z^2 - L1^2) - a1;
    % Yeni düzlemde hedef noktası (x, r)
    dist_sq = x^2 + r^2;
    dist = sqrt(dist_sq);

    % --- 3. DİZ (KNEE) ---
    cos_phi = (L2^2 + L3^2 - dist_sq) / (2 * L2 * L3);
    cos_phi = min(max(cos_phi, -1), 1); % Sayısal koruma
    phi = acos(cos_phi);
    % theta3'ü pozitif yaparsan diz ters yöne kırılır
    theta3_rad = (pi - phi); 

    % --- 4. KALÇA (PITCH) ---
    alpha = atan2(x, r);
    beta = acos((L2^2 + dist_sq - L3^2) / (2 * L2 * dist));
    theta2_rad = alpha + beta;

    % RAD -> DEG
    angles = [theta1_rad; theta2_rad; theta3_rad] * (180/pi);
end

== matlab function Koudruped_simcape/Left Front Step1/MATLAB Function1 ==
  data: t input; pos output; phase_offset input; H_hedef input
function pos = fcn(t, phase_offset, H_hedef)
    pos = zeros(3,1); 
    
    % === 1. ADIM: BU BACAK İÇİN DEĞERLERİ YUKARIDAKİ LİSTEYE GÖRE GİR ===
    X_merkez = 0;       % Ön için 0, Arka için -40
    Y_offset = 44.41;   % Sol için 44.41, Sağ için -44.41
    
    % --- PARAMETRELER ---
    T_kalkis = 2.0;      
    H_baslangic = -190;  
    
    % --- DURUM MAKİNESİ (Sadece Z ekseni hareket eder) ---
    if t < T_kalkis
        z = H_baslangic + (H_hedef - H_baslangic) * (t / T_kalkis);
    else
        z = H_hedef;
    end
    
    x = X_merkez;
    y = Y_offset;
    
    pos = [x; y; z];
end

== matlab function Koudruped_simcape/Left Front Step1/MATLAB Function2 ==
  data: pos input; angles output
function angles = inverse(pos)
    x = pos(1); y = pos(2); z = pos(3);
    
    % --- PARAMETRELER (Senin değerlerin) ---
    L1 = 44.41; a1 = 24.51; L2 = 100; L3 = 100;
    
    % --- 1. OMUZ (ROLL) ---
    theta1_rad = atan2(y, -z) - atan2(L1, sqrt(y^2 + z^2 - L1^2));

    % --- 2. YARDIMCI KOORDİNATLAR ---
    % Bacak düzlemindeki izdüşüm
    r = sqrt(y^2 + z^2 - L1^2) - a1;
    % Yeni düzlemde hedef noktası (x, r)
    dist_sq = x^2 + r^2;
    dist = sqrt(dist_sq);

    % --- 3. DİZ (KNEE) ---
    cos_phi = (L2^2 + L3^2 - dist_sq) / (2 * L2 * L3);
    cos_phi = min(max(cos_phi, -1), 1); % Sayısal koruma
    phi = acos(cos_phi);
    % theta3'ü pozitif yaparsan diz ters yöne kırılır
    theta3_rad = (pi - phi); 

    % --- 4. KALÇA (PITCH) ---
    alpha = atan2(x, r);
    beta = acos((L2^2 + dist_sq - L3^2) / (2 * L2 * dist));
    theta2_rad = alpha + beta;

    % RAD -> DEG
    angles = [theta1_rad; theta2_rad; theta3_rad] * (180/pi);
end

== matlab function Koudruped_simcape/Right Back Step1/MATLAB Function1 ==
  data: t input; pos output; phase_offset input; H_hedef input
function pos = fcn(t, phase_offset, H_hedef)
    pos = zeros(3,1); 
    
    % === 1. ADIM: BU BACAK İÇİN DEĞERLERİ YUKARIDAKİ LİSTEYE GÖRE GİR ===
    X_merkez = -40;       % Ön için 0, Arka için -40
    Y_offset = -44.41;   % Sol için 44.41, Sağ için -44.41
    
    % --- PARAMETRELER ---
    T_kalkis = 2.0;      
    H_baslangic = -190;  
    
    % --- DURUM MAKİNESİ (Sadece Z ekseni hareket eder) ---
    if t < T_kalkis
        z = H_baslangic + (H_hedef - H_baslangic) * (t / T_kalkis);
    else
        z = H_hedef;
    end
    
    x = X_merkez;
    y = Y_offset;
    
    pos = [x; y; z];
end

== matlab function Koudruped_simcape/Right Back Step1/MATLAB Function2 ==
  data: pos input; angles output
function angles = inverse(pos)
    x = pos(1); y = pos(2); z = pos(3);
    
    % --- PARAMETRELER (Senin değerlerin) ---
    L1 = 44.41; a1 = 24.51; L2 = 100; L3 = 100;
    
    % --- 1. OMUZ (ROLL) ---
    % Omuzun dışa doğru açılması için atan2 parametrelerini kontrol et
    % Eğer omuz içeri katlanıyorsa 'y' yerine '-y' deneyebilirsin
    theta1_rad = atan2(y, -z) - atan2(L1, sqrt(y^2 + z^2 - L1^2));

    % --- 2. YARDIMCI KOORDİNATLAR ---
    % Bacak düzlemindeki izdüşüm
    r = sqrt(y^2 + z^2 - L1^2) - a1;
    % Yeni düzlemde hedef noktası (x, r)
    dist_sq = x^2 + r^2;
    dist = sqrt(dist_sq);

    % --- 3. DİZ (KNEE) ---
    cos_phi = (L2^2 + L3^2 - dist_sq) / (2 * L2 * L3);
    cos_phi = min(max(cos_phi, -1), 1); % Sayısal koruma
    phi = acos(cos_phi);
    % theta3'ü pozitif yaparsan diz ters yöne kırılır
    theta3_rad = (pi - phi); 

    % --- 4. KALÇA (PITCH) ---
    alpha = atan2(x, r);
    beta = acos((L2^2 + dist_sq - L3^2) / (2 * L2 * dist));
    theta2_rad = alpha + beta;

    % RAD -> DEG
    angles = [theta1_rad; theta2_rad; theta3_rad] * (180/pi);
end

== matlab function Koudruped_simcape/Right Front Step1/MATLAB Function12 ==
  data: t input; pos output; phase_offset input; H_hedef input
function pos = fcn(t, phase_offset, H_hedef)
    pos = zeros(3,1); 
    
    % === 1. ADIM: BU BACAK İÇİN DEĞERLERİ YUKARIDAKİ LİSTEYE GÖRE GİR ===
    X_merkez = 0;       % Ön için 0, Arka için -40
    Y_offset = -44.41;   % Sol için 44.41, Sağ için -44.41
    
    % --- PARAMETRELER ---
    T_kalkis = 2.0;      
    H_baslangic = -190;  
    
    % --- DURUM MAKİNESİ (Sadece Z ekseni hareket eder) ---
    if t < T_kalkis
        z = H_baslangic + (H_hedef - H_baslangic) * (t / T_kalkis);
    else
        z = H_hedef;
    end
    
    x = X_merkez;
    y = Y_offset;
    
    pos = [x; y; z];
end

== matlab function Koudruped_simcape/Left Front Step/MATLAB Function1 ==
  data: t input; pos output; phase_offset input; H_hedef input
function pos = fcn(t, phase_offset, H_hedef)
    pos = zeros(3,1); 
    
    % --- PARAMETRELER ---
    T_kalkis = 2.0;      
    T_bekleme = 1.0;     
    T_periyot = 1.0;     
    Duty_Factor = 0.5;   
    
    L_adim = 80;         
    H_adim = 30;         
    H_baslangic = -50;   
    Y_offset = 60;       
    
    % --- DURUM MAKİNESİ ---
    if t < T_kalkis
        z = H_baslangic + (H_hedef - H_baslangic) * (t / T_kalkis);
        x = 0;
        pos = [x; Y_offset; z];
        
    elseif t < (T_kalkis + T_bekleme)
        z = H_hedef;
        x = 0;
        pos = [x; Y_offset; z];
        
    else
        t_yurume = t - (T_kalkis + T_bekleme);
        
        % === FADE-IN (YUMUŞAK BAŞLANGIÇ) ÇARPANI ===
        % İlk 2 saniye boyunca adım boyu ve yüksekliği 0'dan 100%'e çıkar
        T_fade = 2.0; 
        k_amp = min(t_yurume / T_fade, 1.0); 
        
        % O anki aktif adım limitleri
        L_aktif = L_adim * k_amp;
        H_aktif = H_adim * k_amp;
        
        t_norm = mod((t_yurume / T_periyot) + phase_offset, 1.0);
        
        if t_norm < Duty_Factor
            % Swing Phase
            t_swing = t_norm / Duty_Factor; 
            x = -(L_aktif/2) + L_aktif * (t_swing - sin(2*pi*t_swing)/(2*pi));
            z = H_hedef + H_aktif * sin(pi * t_swing); 
        else
            % Stance Phase
            t_stance = (t_norm - Duty_Factor) / (1 - Duty_Factor);
            x_start = L_aktif/2;
            x_end = -(L_aktif/2);
            x = x_start + (x_end - x_start) * ((1 - cos(pi * t_stance)) / 2);
            z = H_hedef;
        end
        
        pos = [x; Y_offset; z];
    end
end

== matlab function Koudruped_simcape/Right Front Step1/MATLAB Function13 ==
  data: pos input; angles output
function angles = inverse(pos)
    x = pos(1); y = pos(2); z = pos(3);
    
    % --- PARAMETRELER (Senin değerlerin) ---
    L1 = 44.41; a1 = 24.51; L2 = 100; L3 = 100;
    
    % --- 1. OMUZ (ROLL) ---
    % Omuzun dışa doğru açılması için atan2 parametrelerini kontrol et
    % Eğer omuz içeri katlanıyorsa 'y' yerine '-y' deneyebilirsin
    theta1_rad = atan2(y, -z) - atan2(L1, sqrt(y^2 + z^2 - L1^2));

    % --- 2. YARDIMCI KOORDİNATLAR ---
    % Bacak düzlemindeki izdüşüm
    r = sqrt(y^2 + z^2 - L1^2) - a1;
    % Yeni düzlemde hedef noktası (x, r)
    dist_sq = x^2 + r^2;
    dist = sqrt(dist_sq);

    % --- 3. DİZ (KNEE) ---
    cos_phi = (L2^2 + L3^2 - dist_sq) / (2 * L2 * L3);
    cos_phi = min(max(cos_phi, -1), 1); % Sayısal koruma
    phi = acos(cos_phi);
    % theta3'ü pozitif yaparsan diz ters yöne kırılır
    theta3_rad = (pi - phi); 

    % --- 4. KALÇA (PITCH) ---
    alpha = atan2(x, r);
    beta = acos((L2^2 + dist_sq - L3^2) / (2 * L2 * dist));
    theta2_rad = alpha + beta;

    % RAD -> DEG
    angles = [theta1_rad; theta2_rad; theta3_rad] * (180/pi);
end

== matlab function Koudruped_simcape/Left Back Step2/MATLAB Function1 ==
  data: t input; pos output; phase_offset input; H_hedef input
function pos = fcn(t, phase_offset, H_hedef)
    pos = zeros(3,1); 
    
    % --- PARAMETRELER (Senin Orijinal Değerlerin) ---
    T_kalkis = 2.0;      
    T_bekleme = 1.0;     
    T_periyot = 1.0;     
    Duty_Factor = 0.5;   
    
    L_adim = 80;         
    H_adim = 30;         
    H_baslangic = -50;   
    Y_offset = 60;       
    
    % --- DURUM MAKİNESİ ---
    if t < T_kalkis
        z = H_baslangic + (H_hedef - H_baslangic) * (t / T_kalkis);
        x = 0;
        pos = [x; Y_offset; z];
        
    elseif t < (T_kalkis + T_bekleme)
        z = H_hedef;
        x = 0;
        pos = [x; Y_offset; z];
        
    else
        t_yurume = t - (T_kalkis + T_bekleme);
        
        T_fade = 2.0; 
        k_amp = min(t_yurume / T_fade, 1.0); 
        
        L_aktif = L_adim * k_amp;
        H_aktif = H_adim * k_amp;
        
        t_norm = mod((t_yurume / T_periyot) + phase_offset, 1.0);
        
        if t_norm < Duty_Factor
            % --- SWING PHASE (HAVADA İLERİ ATILMA) ---
            t_swing = t_norm / Duty_Factor; 
            
            x = (L_aktif/2) - L_aktif * (t_swing - sin(2*pi*t_swing)/(2*pi));
            z = H_hedef + H_aktif * sin(pi * t_swing); 
        else
            % --- STANCE PHASE (YERDE İTME) ---
            t_stance = (t_norm - Duty_Factor) / (1 - Duty_Factor);
            
            x_start = -(L_aktif/2);
            x_end = (L_aktif/2);
            x = x_start + (x_end - x_start) * ((1 - cos(pi * t_stance)) / 2);
            z = H_hedef;
        end
        
        pos = [x; Y_offset; z];
    end
end

== matlab function Koudruped_simcape/Left Back Step2/MATLAB Function2 ==
  data: pos input; angles output
function angles = inverse(pos)
    x = pos(1); y = pos(2); z = pos(3);
    
    % --- PARAMETRELER (Senin değerlerin) ---
    L1 = 44.41; a1 = 24.51; L2 = 100; L3 = 100;
    
    % --- 1. OMUZ (ROLL) ---
    theta1_rad = atan2(y, -z) - atan2(L1, sqrt(y^2 + z^2 - L1^2));

    % --- 2. YARDIMCI KOORDİNATLAR ---
    % Bacak düzlemindeki izdüşüm
    r = sqrt(y^2 + z^2 - L1^2) - a1;
    % Yeni düzlemde hedef noktası (x, r)
    dist_sq = x^2 + r^2;
    dist = sqrt(dist_sq);

    % --- 3. DİZ (KNEE) ---
    cos_phi = (L2^2 + L3^2 - dist_sq) / (2 * L2 * L3);
    cos_phi = min(max(cos_phi, -1), 1); % Sayısal koruma
    phi = acos(cos_phi);
    theta3_rad = (pi - phi); 

    % --- 4. KALÇA (PITCH) ---
    alpha = atan2(x, r);
cos_beta = (L2^2 + dist_sq - L3^2) / (2 * L2 * dist);
cos_beta = min(max(cos_beta, -1), 1);  % Sayısal koruma
beta = acos(cos_beta);
    theta2_rad = alpha + beta;

    % RAD -> DEG
    angles = [theta1_rad; theta2_rad; theta3_rad] * (180/pi);
end

== matlab function Koudruped_simcape/Left Front Step2/MATLAB Function1 ==
  data: t input; pos output; phase_offset input; H_hedef input
function pos = fcn(t, phase_offset, H_hedef)
    pos = zeros(3,1); 
    
    % --- PARAMETRELER (Senin Orijinal Değerlerin) ---
    T_kalkis = 2.0;      
    T_bekleme = 1.0;     
    T_periyot = 1.0;     
    Duty_Factor = 0.5;   
    
    L_adim = 80;         
    H_adim = 30;         
    H_baslangic = -50;   
    Y_offset = 60;       
    
    % --- DURUM MAKİNESİ ---
    if t < T_kalkis
        z = H_baslangic + (H_hedef - H_baslangic) * (t / T_kalkis);
        x = 0;
        pos = [x; Y_offset; z];
        
    elseif t < (T_kalkis + T_bekleme)
        z = H_hedef;
        x = 0;
        pos = [x; Y_offset; z];
        
    else
        t_yurume = t - (T_kalkis + T_bekleme);
        
        T_fade = 2.0; 
        k_amp = min(t_yurume / T_fade, 1.0); 
        
        L_aktif = L_adim * k_amp;
        H_aktif = H_adim * k_amp;
        
        t_norm = mod((t_yurume / T_periyot) + phase_offset, 1.0);
        
        if t_norm < Duty_Factor
            % --- SWING PHASE (HAVADA İLERİ ATILMA) ---
            t_swing = t_norm / Duty_Factor; 
            
            x = (L_aktif/2) - L_aktif * (t_swing - sin(2*pi*t_swing)/(2*pi));
            z = H_hedef + H_aktif * sin(pi * t_swing); 
        else
            % --- STANCE PHASE (YERDE İTME) ---
            t_stance = (t_norm - Duty_Factor) / (1 - Duty_Factor);
            
            x_start = -(L_aktif/2);
            x_end = (L_aktif/2);
            x = x_start + (x_end - x_start) * ((1 - cos(pi * t_stance)) / 2);
            z = H_hedef;
        end
        
        pos = [x; Y_offset; z];
    end
end

== matlab function Koudruped_simcape/Left Front Step2/MATLAB Function2 ==
  data: pos input; angles output
function angles = inverse(pos)
    x = pos(1); y = pos(2); z = pos(3);
    
    % --- PARAMETRELER (Senin değerlerin) ---
    L1 = 44.41; a1 = 24.51; L2 = 100; L3 = 100;
    
    % --- 1. OMUZ (ROLL) ---
    theta1_rad = atan2(y, -z) - atan2(L1, sqrt(y^2 + z^2 - L1^2));

    % --- 2. YARDIMCI KOORDİNATLAR ---
    % Bacak düzlemindeki izdüşüm
    r = sqrt(y^2 + z^2 - L1^2) - a1;
    % Yeni düzlemde hedef noktası (x, r)
    dist_sq = x^2 + r^2;
    dist = sqrt(dist_sq);

    % --- 3. DİZ (KNEE) ---
    cos_phi = (L2^2 + L3^2 - dist_sq) / (2 * L2 * L3);
    cos_phi = min(max(cos_phi, -1), 1); % Sayısal koruma
    phi = acos(cos_phi);
    theta3_rad = (pi - phi); 

    % --- 4. KALÇA (PITCH) ---
    alpha = atan2(x, r);
cos_beta = (L2^2 + dist_sq - L3^2) / (2 * L2 * dist);
cos_beta = min(max(cos_beta, -1), 1);  % Sayısal koruma
beta = acos(cos_beta);
    theta2_rad = alpha + beta;

    % RAD -> DEG
    angles = [theta1_rad; theta2_rad; theta3_rad] * (180/pi);
end
